simulink library "casper_library_accumulators"  (Simulink 7.2)
settings: Solver=ode45  SolverMode=SingleTasking  StartTime=0.0  StopTime=10.0  RelTol=1e-3
values from neighbouring files (symbols this model uses):
  blockCountBits = ceil(log2(numBlocks))    [address_gen_vacc_v2_mask.m]
  blockRowBits = 0    [address_gen_vacc_v2_mask.m]
  comp = compi    [bus_accumulator_init.m]    (also in bus_addsub_init.m = comp*2; bus_convert_init.m; bus_logical_init.m = comp*2; bus_maddsub_init.m = max([compa, compb, compc]))
libraries: xbsIndex_r4 x698, xbsReplacements_r4 x61, casper_library_misc x17, xps_library x9
(part 3 of 5)

== system casper_library_accumulators/dram_vacc/ctrl_unit ==
  valid_data : Inport
  sync : Inport  Port=2
  en_RB_addr : Inport  Port=3
  Concat1 : xbsIndex_r4/Concat  num_inputs=3  dbl_ovrd=off  block_type=concat
      settings: block_version=9.2.01
  Convert2 : xbsIndex_r4/Convert  gui_display_data_type=Fixed-point  arith_type=Unsigned  n_bits=30  bin_pt=0  float_type=Single  exp_bits=8  fraction_bits=24  quantization=Truncate  overflow=Wrap  en=off  latency=0  dbl_ovrd=off  pipeline=off  block_type=convert
      settings: xl_area=[0, 0, 0, 0, 0, 0, 0]  block_version=9.2.01
  Delay1 : xbsIndex_r4/Delay  rst=off  infoeditControl=Selection of Reset will increase slice count due to use of real FFs and instead of SRLs  en=off  latency=2  dbl_ovrd=off  reg_retiming=on  block_type=delay
      settings: xl_area=[0, 0, 0, 0, 0, 0, 0]  block_version=9.2.01
  Delay2 : xbsIndex_r4/Delay  rst=off  infoeditControl=Selection of Reset will increase slice count due to use of real FFs and instead of SRLs  en=off  latency=1  dbl_ovrd=off  reg_retiming=on  block_type=delay
      settings: xl_area=[0, 0, 0, 0, 0, 0, 0]  block_version=9.2.01
  Mux : xbsIndex_r4/Mux  inputs=2  en=off  latency=0  precision=Full  arith_type="Signed  (2's comp)"  n_bits=8  bin_pt=2  quantization=Truncate  overflow=Wrap  dbl_ovrd=off  block_type=mux
      settings: xl_area=[0, 0, 0, 0, 0, 0, 0]  block_version=9.2.01
  Mux2 : xbsIndex_r4/Mux  inputs=2  en=off  latency=0  precision=Full  arith_type="Signed  (2's comp)"  n_bits=8  bin_pt=2  quantization=Truncate  overflow=Wrap  dbl_ovrd=off  block_type=mux
      settings: xl_area=[0, 0, 0, 0, 0, 0, 0]  block_version=9.2.01
  RB_active_or_finish : Subsystem
  address_gen_vacc_DRAM : Subsystem  mask{acc_length=acc_length, valid_length=burst_length}
      mask prompts: acc_length "Accumulation length?"; valid_length "Valid period length?"
      mask init:
      | address_gen_vacc_v2_mask;
  cmd_gen : Subsystem
  latch_rb_enable : Subsystem
  negedge : Subsystem
  readback_address_dram_vacc : Subsystem  mask{acc_length=acc_length, valid_length=valid_length}
      mask prompts: acc_length "Accumulation length?"; valid_length "Valid period length?"
      mask init:
      | readback_address_dram_vacc_mask;
  warn period Delay10 : xbsReplacements_r4/Warning  SystemSampleTime=-1  period=1
  warn period Delay20 : xbsReplacements_r4/Warning  SystemSampleTime=-1  period=1
  address : Outport
  cmd_tag : Outport  Port=2
  RB_active : Outport  Port=3
  RWn : Outport  Port=4
  cmd_valid : Outport  Port=5
  ready : Outport  Port=6
  wires:
  latch_rb_enable/2(cmd_tag) -> Concat1/3
  Delay1/1 -> latch_rb_enable/1(sync), readback_address_dram_vacc/1(sync)  "v"
  negedge/1(out) -> latch_rb_enable/3(negedge)
  latch_rb_enable/1(inc_addr_en) -> RB_active_or_finish/1(enable_rb_addr), readback_address_dram_vacc/2(en)
  readback_address_dram_vacc/1(readback_addr) -> Mux2/3
  valid_data/1 -> cmd_gen/1(valid_data)
  cmd_gen/6(rb_addr_en) -> negedge/1(in), Concat1/1, Mux2/1
  cmd_gen/5(ready) -> ready/1
  cmd_gen/4(cmd_valid) -> cmd_valid/1
  cmd_gen/3(RWn) -> Mux/1, RWn/1
  RB_active_or_finish/1(rb_active) -> RB_active/1
  Mux2/1 -> address/1, Convert2/1
  en_RB_addr/1 -> latch_rb_enable/2(rb_addr_enable)
  Delay2/1 -> address_gen_vacc_DRAM/1(sync)
  Concat1/1 -> cmd_tag/1
  Convert2/1 -> Concat1/2
  cmd_gen/2(wr_addr_en) -> address_gen_vacc_DRAM/3(write_en)
  cmd_gen/1(re_addr_en) -> address_gen_vacc_DRAM/2(read_en)
  Mux/1 -> Mux2/2
  address_gen_vacc_DRAM/2(read_addr) -> Mux/3
  address_gen_vacc_DRAM/1(write_addr) -> Mux/2
  sync/1 -> Delay2/1, RB_active_or_finish/2(sync), Delay1/1, cmd_gen/2(sync)

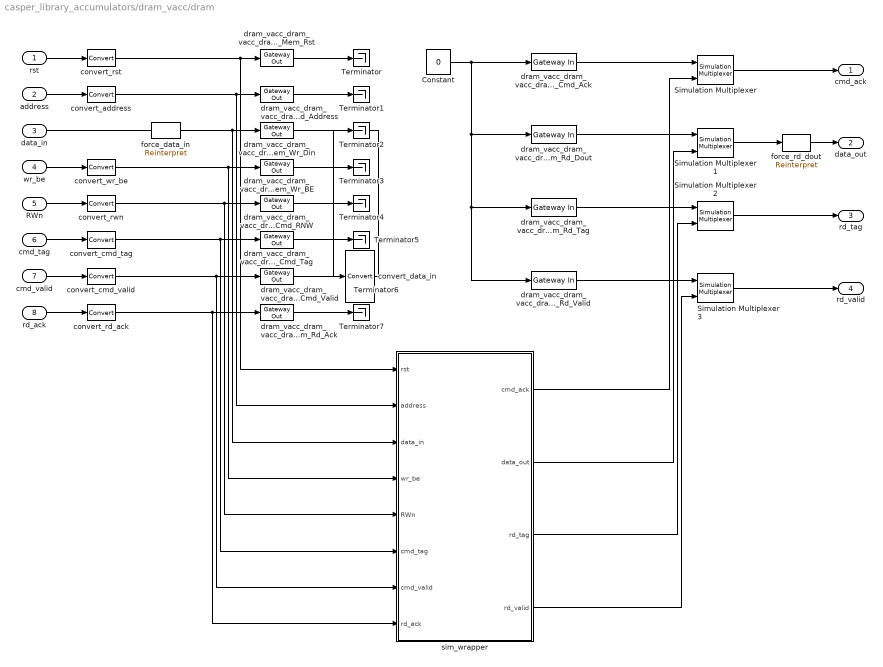
== system casper_library_accumulators/dram_vacc/dram ==
  rst : Inport
  address : Inport  Port=2
  data_in : Inport  Port=3
  wr_be : Inport  Port=4
  RWn : Inport  Port=5
  cmd_tag : Inport  Port=6
  cmd_valid : Inport  Port=7
  rd_ack : Inport  Port=8
  Constant : Constant  Value=0
  Simulation Multiplexer{,1..3} (4 alike) : xbsIndex_r4/Simulation Multiplexer  sim_sel=2  hw_sel=1  block_type=simmux
      settings: infoedit="Distinguish input subsystems as \"simulation only\" and \"generation only\".  The input specified For Simulation will be used during Simulink simulation.  The input specified For Generation will be used during code generation.  This block will typically be used on the output of a HW Co-Simulation, Black Box, or ModelSim subsystem.<P><P>Hardware Notes: This block costs nothing."  block_version=9.2.01
  Terminator{,1..7} (8 alike) : Terminator
  convert_address : xbsIndex_r4/Convert  gui_display_data_type=Fixed-point  arith_type=Unsigned  n_bits=32  bin_pt=0  float_type=Single  exp_bits=8  fraction_bits=24  quantization=Truncate  overflow=Wrap  en=off  latency=0  dbl_ovrd=off  pipeline=off  block_type=convert
      settings: xl_area=[0, 0, 0, 0, 0, 0, 0]  block_version=9.2.01
  convert_cmd_tag : xbsIndex_r4/Convert  gui_display_data_type=Fixed-point  arith_type=Unsigned  n_bits=32  bin_pt=0  float_type=Single  exp_bits=8  fraction_bits=24  quantization=Truncate  overflow=Wrap  en=off  latency=0  dbl_ovrd=off  pipeline=off  block_type=convert
      settings: xl_area=[0, 0, 0, 0, 0, 0, 0]  block_version=9.2.01
  convert_cmd_valid : xbsIndex_r4/Convert  gui_display_data_type=Fixed-point  arith_type=Unsigned  n_bits=1  bin_pt=0  float_type=Single  exp_bits=8  fraction_bits=24  quantization=Truncate  overflow=Wrap  en=off  latency=0  dbl_ovrd=off  pipeline=off  block_type=convert
      settings: xl_area=[0, 0, 0, 0, 0, 0, 0]  block_version=9.2.01
  convert_data_in : xbsIndex_r4/Convert  gui_display_data_type=Fixed-point  arith_type=Unsigned  n_bits=144  bin_pt=0  float_type=Single  exp_bits=8  fraction_bits=24  quantization=Truncate  overflow=Wrap  en=off  latency=0  dbl_ovrd=off  pipeline=off  block_type=convert
      settings: xl_area=[0, 0, 0, 0, 0, 0, 0]  block_version=9.2.01
  convert_rd_ack : xbsIndex_r4/Convert  gui_display_data_type=Fixed-point  arith_type=Unsigned  n_bits=1  bin_pt=0  float_type=Single  exp_bits=8  fraction_bits=24  quantization=Truncate  overflow=Wrap  en=off  latency=0  dbl_ovrd=off  pipeline=off  block_type=convert
      settings: xl_area=[0, 0, 0, 0, 0, 0, 0]  block_version=9.2.01
  convert_rst : xbsIndex_r4/Convert  gui_display_data_type=Fixed-point  arith_type=Unsigned  n_bits=1  bin_pt=0  float_type=Single  exp_bits=8  fraction_bits=24  quantization=Truncate  overflow=Wrap  en=off  latency=0  dbl_ovrd=off  pipeline=off  block_type=convert
      settings: xl_area=[0, 0, 0, 0, 0, 0, 0]  block_version=9.2.01
  convert_rwn : xbsIndex_r4/Convert  gui_display_data_type=Fixed-point  arith_type=Unsigned  n_bits=1  bin_pt=0  float_type=Single  exp_bits=8  fraction_bits=24  quantization=Truncate  overflow=Wrap  en=off  latency=0  dbl_ovrd=off  pipeline=off  block_type=convert
      settings: xl_area=[0, 0, 0, 0, 0, 0, 0]  block_version=9.2.01
  convert_wr_be : xbsIndex_r4/Convert  gui_display_data_type=Fixed-point  arith_type=Unsigned  n_bits=18  bin_pt=0  float_type=Single  exp_bits=8  fraction_bits=24  quantization=Truncate  overflow=Wrap  en=off  latency=0  dbl_ovrd=off  pipeline=off  block_type=convert
      settings: xl_area=[0, 0, 0, 0, 0, 0, 0]  block_version=9.2.01
  dram_vacc_dram_vacc_dram_Mem_Cmd_Ack : xbsIndex_r4/Gateway In  gui_display_data_type=Fixed-point  arith_type=Unsigned  n_bits=1  bin_pt=0  preci_type=Single  exp_width=8  frac_width=24  quantization=Truncate  overflow=Wrap  period=sample_period  dbl_ovrd=off  timing_constraint=None  locs_specified=off  LOCs={}  hdl_port=on  block_type=gatewayin
      settings: infoedit="Gateway in block.  Converts inputs of type Simulink integer, double and fixed point to  Xilinx fixed point type.<P><P>Hardware notes:  In hardware these blocks become top level input ports."  xl_area=[0, 0, 0, 0, 0, 0, 0]  block_version=9.2.01
  dram_vacc_dram_vacc_dram_Mem_Cmd_Address : xbsIndex_r4/Gateway Out  hdl_port=on  timing_constraint=None  locs_specified=off  LOCs={}  block_type=gatewayout
      settings: infoedit="Gateway out block.  Converts Xilinx fixed point inputs into ouputs of type Simulink integer, double, or fixed point.<P><P>Hardware notes:  In hardware these blocks become top level output ports or are discarded, depending on how they are configured."  xl_area=[0, 0, 0, 0, 0, 0, 0]  block_version=9.2.01
  dram_vacc_dram_vacc_dram_Mem_Cmd_RNW : xbsIndex_r4/Gateway Out  hdl_port=on  timing_constraint=None  locs_specified=off  LOCs={}  block_type=gatewayout
      settings: infoedit="Gateway out block.  Converts Xilinx fixed point inputs into ouputs of type Simulink integer, double, or fixed point.<P><P>Hardware notes:  In hardware these blocks become top level output ports or are discarded, depending on how they are configured."  xl_area=[0, 0, 0, 0, 0, 0, 0]  block_version=9.2.01
  dram_vacc_dram_vacc_dram_Mem_Cmd_Tag : xbsIndex_r4/Gateway Out  hdl_port=on  timing_constraint=None  locs_specified=off  LOCs={}  block_type=gatewayout
      settings: infoedit="Gateway out block.  Converts Xilinx fixed point inputs into ouputs of type Simulink integer, double, or fixed point.<P><P>Hardware notes:  In hardware these blocks become top level output ports or are discarded, depending on how they are configured."  xl_area=[0, 0, 0, 0, 0, 0, 0]  block_version=9.2.01
  dram_vacc_dram_vacc_dram_Mem_Cmd_Valid : xbsIndex_r4/Gateway Out  hdl_port=on  timing_constraint=None  locs_specified=off  LOCs={}  block_type=gatewayout
      settings: infoedit="Gateway out block.  Converts Xilinx fixed point inputs into ouputs of type Simulink integer, double, or fixed point.<P><P>Hardware notes:  In hardware these blocks become top level output ports or are discarded, depending on how they are configured."  xl_area=[0, 0, 0, 0, 0, 0, 0]  block_version=9.2.01
  dram_vacc_dram_vacc_dram_Mem_Rd_Ack : xbsIndex_r4/Gateway Out  hdl_port=on  timing_constraint=None  locs_specified=off  LOCs={}  block_type=gatewayout
      settings: infoedit="Gateway out block.  Converts Xilinx fixed point inputs into ouputs of type Simulink integer, double, or fixed point.<P><P>Hardware notes:  In hardware these blocks become top level output ports or are discarded, depending on how they are configured."  xl_area=[0, 0, 0, 0, 0, 0, 0]  block_version=9.2.01
  dram_vacc_dram_vacc_dram_Mem_Rd_Dout : xbsIndex_r4/Gateway In  gui_display_data_type=Fixed-point  arith_type=Unsigned  n_bits=144  bin_pt=0  preci_type=Single  exp_width=8  frac_width=24  quantization=Truncate  overflow=Wrap  period=sample_period  dbl_ovrd=off  timing_constraint=None  locs_specified=off  LOCs={}  hdl_port=on  block_type=gatewayin
      settings: infoedit="Gateway in block.  Converts inputs of type Simulink integer, double and fixed point to  Xilinx fixed point type.<P><P>Hardware notes:  In hardware these blocks become top level input ports."  xl_area=[0, 0, 0, 0, 0, 0, 0]  block_version=9.2.01
  dram_vacc_dram_vacc_dram_Mem_Rd_Tag : xbsIndex_r4/Gateway In  gui_display_data_type=Fixed-point  arith_type=Unsigned  n_bits=32  bin_pt=0  preci_type=Single  exp_width=8  frac_width=24  quantization=Truncate  overflow=Wrap  period=sample_period  dbl_ovrd=off  timing_constraint=None  locs_specified=off  LOCs={}  hdl_port=on  block_type=gatewayin
      settings: infoedit="Gateway in block.  Converts inputs of type Simulink integer, double and fixed point to  Xilinx fixed point type.<P><P>Hardware notes:  In hardware these blocks become top level input ports."  xl_area=[0, 0, 0, 0, 0, 0, 0]  block_version=9.2.01
  dram_vacc_dram_vacc_dram_Mem_Rd_Valid : xbsIndex_r4/Gateway In  gui_display_data_type=Fixed-point  arith_type=Unsigned  n_bits=1  bin_pt=0  preci_type=Single  exp_width=8  frac_width=24  quantization=Truncate  overflow=Wrap  period=sample_period  dbl_ovrd=off  timing_constraint=None  locs_specified=off  LOCs={}  hdl_port=on  block_type=gatewayin
      settings: infoedit="Gateway in block.  Converts inputs of type Simulink integer, double and fixed point to  Xilinx fixed point type.<P><P>Hardware notes:  In hardware these blocks become top level input ports."  xl_area=[0, 0, 0, 0, 0, 0, 0]  block_version=9.2.01
  dram_vacc_dram_vacc_dram_Mem_Rst : xbsIndex_r4/Gateway Out  hdl_port=on  timing_constraint=None  locs_specified=off  LOCs={}  block_type=gatewayout
      settings: infoedit="Gateway out block.  Converts Xilinx fixed point inputs into ouputs of type Simulink integer, double, or fixed point.<P><P>Hardware notes:  In hardware these blocks become top level output ports or are discarded, depending on how they are configured."  xl_area=[0, 0, 0, 0, 0, 0, 0]  block_version=9.2.01
  dram_vacc_dram_vacc_dram_Mem_Wr_BE : xbsIndex_r4/Gateway Out  hdl_port=on  timing_constraint=None  locs_specified=off  LOCs={}  block_type=gatewayout
      settings: infoedit="Gateway out block.  Converts Xilinx fixed point inputs into ouputs of type Simulink integer, double, or fixed point.<P><P>Hardware notes:  In hardware these blocks become top level output ports or are discarded, depending on how they are configured."  xl_area=[0, 0, 0, 0, 0, 0, 0]  block_version=9.2.01
  dram_vacc_dram_vacc_dram_Mem_Wr_Din : xbsIndex_r4/Gateway Out  hdl_port=on  timing_constraint=None  locs_specified=off  LOCs={}  block_type=gatewayout
      settings: infoedit="Gateway out block.  Converts Xilinx fixed point inputs into ouputs of type Simulink integer, double, or fixed point.<P><P>Hardware notes:  In hardware these blocks become top level output ports or are discarded, depending on how they are configured."  xl_area=[0, 0, 0, 0, 0, 0, 0]  block_version=9.2.01
  force_data_in : xbsIndex_r4/Reinterpret  force_arith_type=on  arith_type=Unsigned  force_bin_pt=on  bin_pt=0  block_type=reinterpret
      settings: infoedit="Changes signal type without altering the binary representation.   You can changed the signal between signed and unsigned, and relocate the binary point.<P><P>Hardware notes: In hardware this block costs nothing.<P><P>Example:  Suppose the input is 6 bits wide, signed, with 2 fractional bits, and the output is forced to unsigned with 0 fractional bits.  Then an input of -2.0 (1110.00 in binary 2's complement) becomes an output of 56 (111000 in binary)."  block_version=9.2.01
  force_rd_dout : xbsIndex_r4/Reinterpret  force_arith_type=on  arith_type=Unsigned  force_bin_pt=on  bin_pt=0  block_type=reinterpret
      settings: infoedit="Changes signal type without altering the binary representation.   You can changed the signal between signed and unsigned, and relocate the binary point.<P><P>Hardware notes: In hardware this block costs nothing.<P><P>Example:  Suppose the input is 6 bits wide, signed, with 2 fractional bits, and the output is forced to unsigned with 0 fractional bits.  Then an input of -2.0 (1110.00 in binary 2's complement) becomes an output of 56 (111000 in binary)."  block_version=9.2.01
  sim_wrapper : Subsystem
  cmd_ack : Outport
  data_out : Outport  Port=2
  rd_tag : Outport  Port=3
  rd_valid : Outport  Port=4
  wires:
  force_rd_dout/1 -> data_out/1
  force_data_in/1 -> dram_vacc_dram_vacc_dram_Mem_Wr_Din/1, sim_wrapper/3(data_in)
  convert_rd_ack/1 -> dram_vacc_dram_vacc_dram_Mem_Rd_Ack/1, sim_wrapper/8(rd_ack)
  convert_cmd_valid/1 -> dram_vacc_dram_vacc_dram_Mem_Cmd_Valid/1, sim_wrapper/7(cmd_valid)
  convert_cmd_tag/1 -> dram_vacc_dram_vacc_dram_Mem_Cmd_Tag/1, sim_wrapper/6(cmd_tag)
  convert_rwn/1 -> dram_vacc_dram_vacc_dram_Mem_Cmd_RNW/1, sim_wrapper/5(RWn)
  convert_wr_be/1 -> dram_vacc_dram_vacc_dram_Mem_Wr_BE/1, sim_wrapper/4(wr_be)
  convert_data_in/1 -> force_data_in/1
  convert_address/1 -> dram_vacc_dram_vacc_dram_Mem_Cmd_Address/1, sim_wrapper/2(address)
  convert_rst/1 -> dram_vacc_dram_vacc_dram_Mem_Rst/1, sim_wrapper/1(rst)
  rd_ack/1 -> convert_rd_ack/1
  cmd_valid/1 -> convert_cmd_valid/1
  cmd_tag/1 -> convert_cmd_tag/1
  RWn/1 -> convert_rwn/1
  data_in/1 -> convert_data_in/1
  rst/1 -> convert_rst/1
  address/1 -> convert_address/1
  wr_be/1 -> convert_wr_be/1
  dram_vacc_dram_vacc_dram_Mem_Rst/1 -> Terminator/1
  dram_vacc_dram_vacc_dram_Mem_Cmd_Address/1 -> Terminator1/1
  dram_vacc_dram_vacc_dram_Mem_Wr_Din/1 -> Terminator2/1
  dram_vacc_dram_vacc_dram_Mem_Wr_BE/1 -> Terminator3/1
  dram_vacc_dram_vacc_dram_Mem_Cmd_RNW/1 -> Terminator4/1
  dram_vacc_dram_vacc_dram_Mem_Cmd_Tag/1 -> Terminator5/1
  dram_vacc_dram_vacc_dram_Mem_Cmd_Valid/1 -> Terminator6/1
  dram_vacc_dram_vacc_dram_Mem_Rd_Ack/1 -> Terminator7/1
  Constant/1 -> dram_vacc_dram_vacc_dram_Mem_Cmd_Ack/1, dram_vacc_dram_vacc_dram_Mem_Rd_Dout/1, dram_vacc_dram_vacc_dram_Mem_Rd_Tag/1, dram_vacc_dram_vacc_dram_Mem_Rd_Valid/1
  dram_vacc_dram_vacc_dram_Mem_Cmd_Ack/1 -> Simulation Multiplexer/1
  Simulation Multiplexer/1 -> cmd_ack/1
  dram_vacc_dram_vacc_dram_Mem_Rd_Dout/1 -> Simulation Multiplexer1/1
  Simulation Multiplexer1/1 -> force_rd_dout/1
  Simulation Multiplexer2/1 -> rd_tag/1
  Simulation Multiplexer3/1 -> rd_valid/1
  dram_vacc_dram_vacc_dram_Mem_Rd_Tag/1 -> Simulation Multiplexer2/1
  dram_vacc_dram_vacc_dram_Mem_Rd_Valid/1 -> Simulation Multiplexer3/1
  sim_wrapper/1(cmd_ack) -> Simulation Multiplexer/2
  sim_wrapper/2(data_out) -> Simulation Multiplexer1/2
  sim_wrapper/3(rd_tag) -> Simulation Multiplexer2/2
  sim_wrapper/4(rd_valid) -> Simulation Multiplexer3/2

== system casper_library_accumulators/dram_vacc/fifo_empty_check ==
  cmd_valid : Inport
  tag_in : Inport  Port=2
  RWn : Inport  Port=3
  dram_data_tag : Inport  Port=4
  rd_ack : Inport  Port=5
  rd_valid : Inport  Port=6
  Convert : xbsIndex_r4/Convert  gui_display_data_type=Fixed-point  arith_type=Boolean  n_bits=8  bin_pt=6  float_type=Single  exp_bits=8  fraction_bits=24  quantization=Truncate  overflow=Wrap  en=off  latency=0  dbl_ovrd=off  pipeline=off  block_type=convert
      settings: xl_area=[0, 0, 0, 0, 0, 0, 0]  block_version=9.2.01
  Counter : xbsIndex_r4/Counter  cnt_type=Free Running  cnt_to=Inf  operation=Up  start_count=0  cnt_by_val=1  arith_type=Unsigned  n_bits=1  bin_pt=0  load_pin=off  rst=off  en=on  explicit_period=off  period=1  dbl_ovrd=off  use_behavioral_HDL=on  implementation=Fabric  use_rpm=on  block_type=counter
      settings: xl_area=[0, 0, 0, 0, 0, 0, 0]  block_version=9.2.01
  Delay1 : xbsIndex_r4/Delay  rst=off  infoeditControl=Selection of Reset will increase slice count due to use of real FFs and instead of SRLs  en=off  latency=1  dbl_ovrd=off  reg_retiming=on  block_type=delay
      settings: xl_area=[0, 0, 0, 0, 0, 0, 0]  block_version=9.2.01
  Delay2 : xbsIndex_r4/Delay  rst=off  infoeditControl=Selection of Reset will increase slice count due to use of real FFs and instead of SRLs  en=off  latency=1  dbl_ovrd=off  reg_retiming=on  block_type=delay
      settings: xl_area=[0, 0, 0, 0, 0, 0, 0]  block_version=9.2.01
  Logical : xbsIndex_r4/Logical  logical_function=AND  inputs=2  en=off  latency=0  precision=Full  arith_type=Unsigned  n_bits=8  bin_pt=2  align_bp=on  dbl_ovrd=off  block_type=logical
      settings: xl_area=[0, 0, 0, 0, 0, 0, 0]  block_version=9.2.01
  Logical1 : xbsIndex_r4/Logical  logical_function=AND  inputs=3  en=off  latency=0  precision=Full  arith_type=Unsigned  n_bits=8  bin_pt=2  align_bp=on  dbl_ovrd=off  block_type=logical
      settings: xl_area=[0, 0, 0, 0, 0, 0, 0]  block_version=9.2.01
  Logical2 : xbsIndex_r4/Logical  logical_function=AND  inputs=2  en=off  latency=0  precision=Full  arith_type=Unsigned  n_bits=8  bin_pt=2  align_bp=on  dbl_ovrd=off  block_type=logical
      settings: xl_area=[0, 0, 0, 0, 0, 0, 0]  block_version=9.2.01
  Register1 : xbsIndex_r4/Register  init=0  rst=on  en=on  dbl_ovrd=off  block_type=register
      settings: xl_area=[0, 0, 0, 0, 0, 0, 0]  block_version=9.2.01
  Relational : xbsIndex_r4/Relational  mode=a=b  en=off  latency=1  dbl_ovrd=off  block_type=relational
      settings: xl_area=[0, 0, 0, 0, 0, 0, 0]  block_version=9.2.01
  Relational1 : xbsIndex_r4/Relational  mode=a!=b  en=on  latency=1  dbl_ovrd=off  block_type=relational
      settings: xl_area=[0, 0, 0, 0, 0, 0, 0]  block_version=9.2.01
  last_read_tag : xbsIndex_r4/Register  init=0  rst=off  en=on  dbl_ovrd=off  block_type=register
      settings: xl_area=[0, 0, 0, 0, 0, 0, 0]  block_version=9.2.01
  negedge : Subsystem
  warn period Logical10 : xbsReplacements_r4/Warning  SystemSampleTime=-1  period=1
  warn period Register10 : xbsReplacements_r4/Warning  SystemSampleTime=-1  period=1
  warn period Relational10 : xbsReplacements_r4/Warning  SystemSampleTime=-1  period=1
  done : Outport
  wires:
  Logical2/1 -> Register1/2
  Convert/1 -> Register1/1, Register1/3
  Register1/1 -> done/1
  negedge/1(out) -> Convert/1
  Relational1/1 -> Logical2/1
  Counter/1 -> negedge/1(in)
  Logical1/1 -> Counter/1
  Relational/1 -> Logical1/1
  Delay1/1 -> Logical1/2
  rd_ack/1 -> Delay1/1
  Delay2/1 -> Logical1/3
  rd_valid/1 -> Delay2/1
  dram_data_tag/1 -> Relational/2
  last_read_tag/1 -> Relational/1, Relational1/2
  Logical/1 -> last_read_tag/2, Logical2/2, Relational1/3
  tag_in/1 -> last_read_tag/1, Relational1/1
  RWn/1 -> Logical/2
  cmd_valid/1 -> Logical/1

== system casper_library_accumulators/dsp48e_bram_vacc/delay_bram ==
  In1 : Inport
  Constant2 : xbsIndex_r4/Constant  const=1  gui_display_data_type=Fixed-point  arith_type=Boolean  n_bits=1  bin_pt=0  preci_type=Single  exp_width=8  frac_width=24  explicit_period=on  period=1  equ=P=C  opselect=C  inp2=PCIN>>17  opr=+  inp1=P  carry=CIN  dbl_ovrd=off  block_type=constant
  Counter : xbsIndex_r4/Counter  cnt_type=Count Limited  cnt_to=DelayLen - bram_latency - 1  operation=Up  start_count=0  cnt_by_val=1  arith_type=Unsigned  n_bits=BitWidth  bin_pt=0  load_pin=off  rst=off  en=off  explicit_period=off  period=1  dbl_ovrd=off  use_behavioral_HDL=on  implementation=Fabric  use_rpm=off  block_type=counter
      settings: xl_area=[0, 0, 0, 0, 0, 0, 0]
  Single Port RAM : xbsIndex_r4/Single Port RAM  depth=2^BitWidth  initVector=0  distributed_mem=Block RAM  write_mode=Read Before Write  rst=off  init_reg=0  en=off  latency=bram_latency  dbl_ovrd=off  optimize=Area  use_rpm=off  block_type=spram
      settings: xl_area=[0, 0, 0, 0, 0, 0, 0]  block_version=10.1.3
  Out1 : Outport
  wires:
  Single Port RAM/1 -> Out1/1
  Counter/1 -> Single Port RAM/1
  In1/1 -> Single Port RAM/2
  Constant2/1 -> Single Port RAM/3

== system casper_library_accumulators/dsp48e_bram_vacc/pulse_ext ==
  in : Inport
  Constant5 : xbsIndex_r4/Constant  const=pulse_len  gui_display_data_type=Fixed-point  arith_type=Unsigned  n_bits=bits  bin_pt=0  preci_type=Single  exp_width=8  frac_width=24  explicit_period=off  period=1  equ=P=C  opselect=C  inp2=PCIN>>17  opr=+  inp1=P  carry=CIN  dbl_ovrd=off  block_type=constant
  Counter3 : xbsIndex_r4/Counter  cnt_type=Free Running  cnt_to=1023  operation=Up  start_count=0  cnt_by_val=1  arith_type=Unsigned  n_bits=bits  bin_pt=0  load_pin=off  rst=on  en=on  explicit_period=on  period=1  dbl_ovrd=off  use_behavioral_HDL=on  implementation=Fabric  use_rpm=on  block_type=counter
      settings: xl_area=[0, 0, 0, 0, 0, 0, 0]
  Relational5 : xbsIndex_r4/Relational  mode=a!=b  en=off  latency=0  dbl_ovrd=off  block_type=relational
      settings: xl_area=[0, 0, 0, 0, 0, 0, 0]  block_version=10.1.3
  posedge : Subsystem  Tag=Rising Edge Detector
  out : Outport
  wires:
  posedge/1(Out) -> Counter3/1
  in/1 -> posedge/1(In)
  Relational5/1 -> out/1, Counter3/2
  Constant5/1 -> Relational5/2
  Counter3/1 -> Relational5/1

== system casper_library_accumulators/qdr_vacc/acc ==
  a : Inport
  b : Inport  Port=2
  blank_b : Inport  Port=3
  AddSub4 : xbsIndex_r4/AddSub  mode=Addition  use_carryin=off  use_carryout=off  en=off  latency=2  precision=User Defined  arith_type="Signed  (2's comp)"  n_bits=4  bin_pt=0  quantization="Round  (unbiased: +/- Inf)"  overflow=Wrap  dbl_ovrd=off  use_behavioral_HDL=on  hw_selection=Fabric  pipelined=on  use_rpm=on  block_type=addsub
      settings: xl_area=[0, 0, 0, 0, 0, 0, 0]  block_version=9.2.01
  AddSub5 : xbsIndex_r4/AddSub  mode=Addition  use_carryin=off  use_carryout=off  en=off  latency=2  precision=User Defined  arith_type="Signed  (2's comp)"  n_bits=32  bin_pt=0  quantization="Round  (unbiased: +/- Inf)"  overflow=Wrap  dbl_ovrd=off  use_behavioral_HDL=on  hw_selection=Fabric  pipelined=on  use_rpm=on  block_type=addsub
      settings: xl_area=[0, 0, 0, 0, 0, 0, 0]  block_version=9.2.01
  Concat1v1 : xbsIndex_r4/Concat  num_inputs=2  dbl_ovrd=off  block_type=concat
      settings: block_version=9.2.01
  Constant3 : xbsIndex_r4/Constant  const=0  gui_display_data_type=Fixed-point  arith_type=Unsigned  n_bits=36  bin_pt=0  preci_type=Single  exp_width=8  frac_width=24  explicit_period=on  period=1  equ=P=C  opselect=C  inp2=PCIN>>17  opr=+  inp1=P  carry=CIN  dbl_ovrd=off  block_type=constant
      settings: block_version=9.2.01
  Reinterpret{,1,4..5} (4 alike) : xbsIndex_r4/Reinterpret  force_arith_type=on  arith_type="Signed  (2's comp)"  force_bin_pt=on  bin_pt=0  block_type=reinterpret
      settings: infoedit="Changes signal type without altering the binary representation.   You can changed the signal between signed and unsigned, and relocate the binary point.<P><P>Hardware notes: In hardware this block costs nothing.<P><P>Example:  Suppose the input is 6 bits wide, signed, with 2 fractional bits, and the output is forced to unsigned with 0 fractional bits.  Then an input of -2.0 (1110.00 in binary 2's complement) becomes an output of 56 (111000 in binary)."  block_version=9.2.01
  Reinterpret8 : xbsIndex_r4/Reinterpret  force_arith_type=on  arith_type=Unsigned  force_bin_pt=on  bin_pt=0  block_type=reinterpret
      settings: infoedit="Changes signal type without altering the binary representation.   You can changed the signal between signed and unsigned, and relocate the binary point.<P><P>Hardware notes: In hardware this block costs nothing.<P><P>Example:  Suppose the input is 6 bits wide, signed, with 2 fractional bits, and the output is forced to unsigned with 0 fractional bits.  Then an input of -2.0 (1110.00 in binary 2's complement) becomes an output of 56 (111000 in binary)."  block_version=9.2.01
  Reinterpret9 : xbsIndex_r4/Reinterpret  force_arith_type=on  arith_type=Unsigned  force_bin_pt=on  bin_pt=0  block_type=reinterpret
      settings: infoedit="Changes signal type without altering the binary representation.   You can changed the signal between signed and unsigned, and relocate the binary point.<P><P>Hardware notes: In hardware this block costs nothing.<P><P>Example:  Suppose the input is 6 bits wide, signed, with 2 fractional bits, and the output is forced to unsigned with 0 fractional bits.  Then an input of -2.0 (1110.00 in binary 2's complement) becomes an output of 56 (111000 in binary)."  block_version=9.2.01
  Slice1 : xbsIndex_r4/Slice  nbits=4  boolean_output=off  mode=Lower Bit Location + Width  bit1=96  base1=MSB of Input  bit0=32  base0=LSB of Input  dbl_ovrd=off  block_type=slice
      settings: infoedit="Extracts a given range of bits from each input sample and presents it at the output.  The output type is ordinarily unsigned with binary point at zero, but can be Boolean when the slice is one bit wide.<P><P>Hardware notes: In hardware this block costs nothing."  block_version=9.2.01
  Slice15 : xbsIndex_r4/Slice  nbits=4  boolean_output=off  mode=Lower Bit Location + Width  bit1=96  base1=MSB of Input  bit0=32  base0=LSB of Input  dbl_ovrd=off  block_type=slice
      settings: infoedit="Extracts a given range of bits from each input sample and presents it at the output.  The output type is ordinarily unsigned with binary point at zero, but can be Boolean when the slice is one bit wide.<P><P>Hardware notes: In hardware this block costs nothing."  block_version=9.2.01
  Slice16 : xbsIndex_r4/Slice  nbits=32  boolean_output=off  mode=Lower Bit Location + Width  bit1=-32  base1=MSB of Input  bit0=0  base0=LSB of Input  dbl_ovrd=off  block_type=slice
      settings: infoedit="Extracts a given range of bits from each input sample and presents it at the output.  The output type is ordinarily unsigned with binary point at zero, but can be Boolean when the slice is one bit wide.<P><P>Hardware notes: In hardware this block costs nothing."  block_version=9.2.01
  Slice2 : xbsIndex_r4/Slice  nbits=32  boolean_output=off  mode=Lower Bit Location + Width  bit1=-32  base1=MSB of Input  bit0=0  base0=LSB of Input  dbl_ovrd=off  block_type=slice
      settings: infoedit="Extracts a given range of bits from each input sample and presents it at the output.  The output type is ordinarily unsigned with binary point at zero, but can be Boolean when the slice is one bit wide.<P><P>Hardware notes: In hardware this block costs nothing."  block_version=9.2.01
  rd_addr_sel : xbsIndex_r4/Mux  inputs=2  en=off  latency=0  precision=Full  arith_type=Unsigned  n_bits=16  bin_pt=14  quantization=Truncate  overflow=Wrap  dbl_ovrd=off  block_type=mux
  Out : Outport
  wires:
  Constant3/1 -> rd_addr_sel/3
  blank_b/1 -> rd_addr_sel/1
  rd_addr_sel/1 -> Slice1/1, Slice2/1
  b/1 -> rd_addr_sel/2
  AddSub5/1 -> Reinterpret9/1
  Reinterpret5/1 -> AddSub5/2
  Slice2/1 -> Reinterpret5/1
  Slice16/1 -> Reinterpret1/1
  Reinterpret1/1 -> AddSub5/1
  Reinterpret9/1 -> Concat1v1/2
  Concat1v1/1 -> Out/1
  a/1 -> Slice16/1, Slice15/1
  AddSub4/1 -> Reinterpret8/1
  Reinterpret4/1 -> AddSub4/2
  Slice1/1 -> Reinterpret4/1
  Slice15/1 -> Reinterpret/1
  Reinterpret/1 -> AddSub4/1
  Reinterpret8/1 -> Concat1v1/1

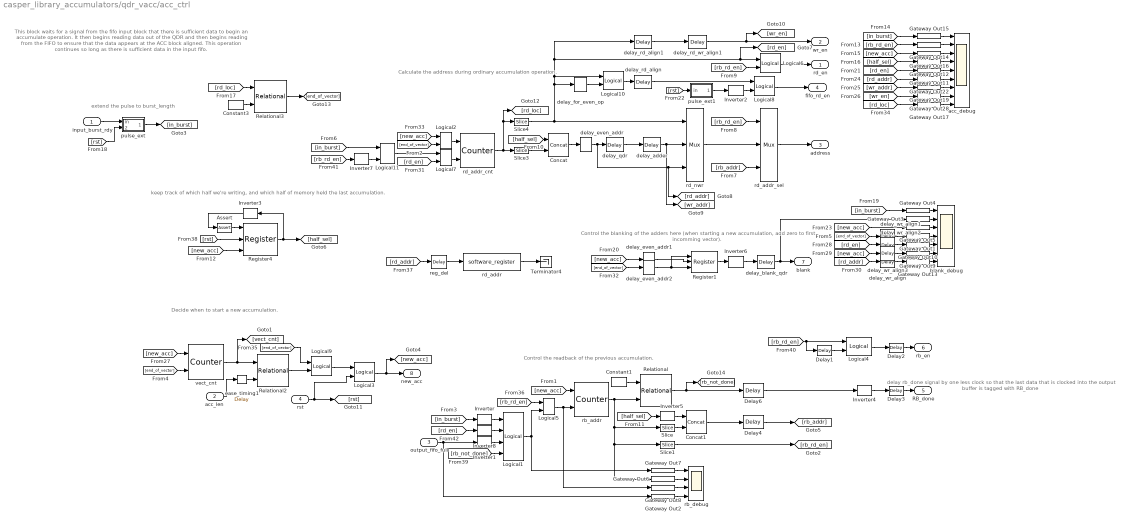
== system casper_library_accumulators/qdr_vacc/acc_ctrl ==
  note: extend the pulse to
      | burst_length
  note: This block waits for a signal from the
      | fifo input block that there is sufficient data
      | to begin an accumulate operation.
      |
      | It then begins reading data out of the QDR and
      | then begins reading from the FIFO to ensure
      | that the data appears at the ACC block aligned.
      |
      | This operation continues so long as there is
      | sufficient data in the input fifo.
  note: keep track of which half we're writing,
      | and which half of memory
      | held the last accumulation.
  note: delay rb_done signal by
      | one less clock so that the last
      | data that is clocked into
      | the output buffer is tagged with RB_done
  note: Control the readback of the
      | previous accumulation.
  note: Control the blanking of the
      | adders here (when starting a
      | new accumulation, add zero
      | to first incomming vector).
  note: Calculate the address during ordinary
      | accumulation operation.
  note: Decide when to start a new accumulation.
  input_burst_rdy : Inport
  acc_len : Inport  Port=2
  output_fifo_full : Inport  Port=3
  rst : Inport  Port=4
  Assert : xbsIndex_r4/Assert  assert_type=on  type_source=Explicitly  gui_display_data_type=Fixed-point  arith_type=Unsigned  n_bits=1  bin_pt=0  preci_type=Single  exp_width=8  frac_width=24  assert_rate=on  rate_source=Explicitly  period=1  output_port=on  block_type=assert
      settings: infoedit=Asserts a user-defined sample rate and/or type on a signal.<P><P>Hardware notes: In hardware this block costs nothing.  block_version=10.1.3
  Concat : xbsIndex_r4/Concat  num_inputs=2  dbl_ovrd=off  block_type=concat
      settings: block_version=10.1.3
  Concat1 : xbsIndex_r4/Concat  num_inputs=2  dbl_ovrd=off  block_type=concat
      settings: block_version=10.1.3
  Constant1 : xbsIndex_r4/Constant  const=vector_len - 1  gui_display_data_type=Fixed-point  arith_type=Unsigned  n_bits=vector_bits  bin_pt=0  preci_type=Single  exp_width=8  frac_width=24  explicit_period=on  period=1  equ=P=C  opselect=C  inp2=PCIN>>17  opr=+  inp1=P  carry=CIN  dbl_ovrd=off  block_type=constant
  Constant3 : xbsIndex_r4/Constant  const=vector_len-1  gui_display_data_type=Fixed-point  arith_type=Unsigned  n_bits=vector_bits  bin_pt=0  preci_type=Single  exp_width=8  frac_width=24  explicit_period=on  period=1  equ=P=C  opselect=C  inp2=PCIN>>17  opr=+  inp1=P  carry=CIN  dbl_ovrd=off  block_type=constant
  Delay1 : xbsIndex_r4/Delay  rst=off  infoeditControl=Selection of Reset will increase slice count due to use of real FFs and instead of SRLs  en=off  latency=1  dbl_ovrd=off  reg_retiming=on  block_type=delay
  Delay2 : xbsIndex_r4/Delay  rst=off  infoeditControl=Selection of Reset will increase slice count due to use of real FFs and instead of SRLs  en=off  latency=delay_qdr  dbl_ovrd=off  reg_retiming=on  block_type=delay
  Delay3 : xbsIndex_r4/Delay  rst=off  infoeditControl=Selection of Reset will increase slice count due to use of real FFs and instead of SRLs  en=off  latency=delay_qdr-1  dbl_ovrd=off  reg_retiming=on  block_type=delay
  Delay4 : xbsIndex_r4/Delay  rst=off  infoeditControl=Selection of Reset will increase slice count due to use of real FFs and instead of SRLs  en=off  latency=1  dbl_ovrd=off  reg_retiming=on  block_type=delay
  Delay6 : xbsIndex_r4/Delay  rst=off  infoeditControl=Selection of Reset will increase slice count due to use of real FFs and instead of SRLs  en=off  latency=1  dbl_ovrd=off  reg_retiming=on  block_type=delay
  Gateway Out{1..17,19,22,28} (20 alike) : xbsIndex_r4/Gateway Out  hdl_port=off  timing_constraint=None  locs_specified=off  LOCs={}  block_type=gatewayout
      settings: infoedit="Gateway out block.  Converts Xilinx fixed point inputs into ouputs of type Simulink integer, double, or fixed point.<P><P>Hardware notes:  In hardware these blocks become top level output ports or are discarded, depending on how they are configured."  xl_area=[0, 0, 0, 0, 0, 0, 0]  block_version=10.1.3
  Inverter{,1..2,4..8} (8 alike) : xbsIndex_r4/Inverter  en=off  latency=0  dbl_ovrd=off  block_type=inv
  Inverter3 : xbsIndex_r4/Inverter  Orientation=left  en=off  latency=0  dbl_ovrd=off  block_type=inv
  Logical1 : xbsIndex_r4/Logical  logical_function=AND  inputs=4  en=off  latency=0  precision=Full  arith_type=Unsigned  n_bits=16  bin_pt=0  align_bp=on  dbl_ovrd=off  block_type=logical
  Logical{2..7,10} (7 alike) : xbsIndex_r4/Logical  logical_function=OR  inputs=2  en=off  latency=0  precision=Full  arith_type=Unsigned  n_bits=16  bin_pt=0  align_bp=on  dbl_ovrd=off  block_type=logical
  Logical11 : xbsIndex_r4/Logical  logical_function=AND  inputs=2  en=off  latency=0  precision=Full  arith_type=Unsigned  n_bits=16  bin_pt=0  align_bp=on  dbl_ovrd=off  block_type=logical
  Logical8 : xbsIndex_r4/Logical  logical_function=AND  inputs=2  en=off  latency=0  precision=Full  arith_type=Unsigned  n_bits=16  bin_pt=0  align_bp=on  dbl_ovrd=off  block_type=logical
  Logical9 : xbsIndex_r4/Logical  logical_function=AND  inputs=2  en=off  latency=0  precision=Full  arith_type=Unsigned  n_bits=16  bin_pt=0  align_bp=on  dbl_ovrd=off  block_type=logical
  Register1 : xbsIndex_r4/Register  init=0  rst=on  en=on  dbl_ovrd=off  block_type=register
  Register4 : xbsIndex_r4/Register  init=0  rst=on  en=on  dbl_ovrd=off  block_type=register
  Relational : xbsIndex_r4/Relational  mode=a>=b  en=off  latency=0  dbl_ovrd=off  block_type=relational
      settings: block_version=10.1.3
  Relational2 : xbsIndex_r4/Relational  mode=a>=b  en=off  latency=0  dbl_ovrd=off  block_type=relational
      settings: block_version=10.1.3
  Relational3 : xbsIndex_r4/Relational  mode=a>=b  en=off  latency=0  dbl_ovrd=off  block_type=relational
      settings: block_version=10.1.3
  Slice : xbsIndex_r4/Slice  nbits=vector_bits-1  boolean_output=off  mode=Lower Bit Location + Width  bit1=0  base1=MSB of Input  bit0=1  base0=LSB of Input  dbl_ovrd=off  block_type=slice
      settings: infoedit="Extracts a given range of bits from each input sample and presents it at the output.  The output type is ordinarily unsigned with binary point at zero, but can be Boolean when the slice is one bit wide.<P><P>Hardware notes: In hardware this block costs nothing."  block_version=10.1.3
  Slice1 : xbsIndex_r4/Slice  nbits=1  boolean_output=on  mode=Lower Bit Location + Width  bit1=-1  base1=MSB of Input  bit0=0  base0=LSB of Input  dbl_ovrd=off  block_type=slice
      settings: infoedit="Extracts a given range of bits from each input sample and presents it at the output.  The output type is ordinarily unsigned with binary point at zero, but can be Boolean when the slice is one bit wide.<P><P>Hardware notes: In hardware this block costs nothing."  block_version=10.1.3
  Slice3 : xbsIndex_r4/Slice  nbits=1  boolean_output=off  mode=Two Bit Locations  bit1=0  base1=MSB of Input  bit0=1  base0=LSB of Input  dbl_ovrd=off  block_type=slice
      settings: infoedit="Extracts a given range of bits from each input sample and presents it at the output.  The output type is ordinarily unsigned with binary point at zero, but can be Boolean when the slice is one bit wide.<P><P>Hardware notes: In hardware this block costs nothing."  block_version=10.1.3
  Slice4 : xbsIndex_r4/Slice  nbits=1  boolean_output=on  mode=Lower Bit Location + Width  bit1=-1  base1=MSB of Input  bit0=0  base0=LSB of Input  dbl_ovrd=off  block_type=slice
      settings: infoedit="Extracts a given range of bits from each input sample and presents it at the output.  The output type is ordinarily unsigned with binary point at zero, but can be Boolean when the slice is one bit wide.<P><P>Hardware notes: In hardware this block costs nothing."  block_version=10.1.3
  Terminator4 : Terminator
  acc_debug : Scope  NumInputPorts=9
      settings: TimeRange=10000  YMin=0~-1~-1~0.95~0~500~500~0~-5  YMax=1~1~1~1.05~1~1100~1100~1~5  SaveName=ScopeData5
  blank_debug : Scope  NumInputPorts=7
      settings: TimeRange=10000  YMin=0~1~-1~-1~0~-1~50  YMax=1~1~1~1~1~1~250  SaveName=ScopeData6
  delay_adder : xbsIndex_r4/Delay  rst=off  infoeditControl=Selection of Reset will increase slice count due to use of real FFs and instead of SRLs  en=off  latency=delay_adder  dbl_ovrd=off  reg_retiming=on  block_type=delay
  delay_blank_qdr : xbsIndex_r4/Delay  rst=off  infoeditControl=Selection of Reset will increase slice count due to use of real FFs and instead of SRLs  en=off  latency=delay_qdr  dbl_ovrd=off  reg_retiming=on  block_type=delay
  delay_even_addr : xbsIndex_r4/Delay  rst=off  infoeditControl=Selection of Reset will increase slice count due to use of real FFs and instead of SRLs  en=off  latency=1  dbl_ovrd=off  reg_retiming=on  block_type=delay
  delay_even_addr1 : xbsIndex_r4/Delay  rst=off  infoeditControl=Selection of Reset will increase slice count due to use of real FFs and instead of SRLs  en=off  latency=1  dbl_ovrd=off  reg_retiming=on  block_type=delay
  delay_even_addr2 : xbsIndex_r4/Delay  rst=off  infoeditControl=Selection of Reset will increase slice count due to use of real FFs and instead of SRLs  en=off  latency=1  dbl_ovrd=off  reg_retiming=on  block_type=delay
  delay_for_even_op : xbsIndex_r4/Delay  rst=off  infoeditControl=Selection of Reset will increase slice count due to use of real FFs and instead of SRLs  en=off  latency=1  dbl_ovrd=off  reg_retiming=on  block_type=delay
  delay_qdr : xbsIndex_r4/Delay  rst=off  infoeditControl=Selection of Reset will increase slice count due to use of real FFs and instead of SRLs  en=off  latency=delay_qdr  dbl_ovrd=off  reg_retiming=on  block_type=delay
  delay_rd_align : xbsIndex_r4/Delay  rst=off  infoeditControl=Selection of Reset will increase slice count due to use of real FFs and instead of SRLs  en=off  latency=delay_qdr-delay_in_fifo  dbl_ovrd=off  reg_retiming=on  block_type=delay
  delay_rd_align1 : xbsIndex_r4/Delay  rst=off  infoeditControl=Selection of Reset will increase slice count due to use of real FFs and instead of SRLs  en=off  latency=delay_qdr  dbl_ovrd=off  reg_retiming=on  block_type=delay
  delay_rd_wr_align1 : xbsIndex_r4/Delay  rst=off  infoeditControl=Selection of Reset will increase slice count due to use of real FFs and instead of SRLs  en=off  latency=delay_adder  dbl_ovrd=off  reg_retiming=on  block_type=delay
  delay_wr_align{,1..3} (4 alike) : xbsIndex_r4/Delay  rst=off  infoeditControl=Selection of Reset will increase slice count due to use of real FFs and instead of SRLs  en=off  latency=delay_qdr  dbl_ovrd=off  reg_retiming=on  block_type=delay
  ease_timing1 : xbsIndex_r4/Delay  rst=off  infoeditControl=Selection of Reset will increase slice count due to use of real FFs and instead of SRLs  en=off  latency=1  dbl_ovrd=off  reg_retiming=on  block_type=delay
  pulse_ext : Subsystem  AncestorBlock=casper_library_misc/pulse_ext  mask(pulse_ext){pulse_len=burst_len}
      mask prompts: pulse_len "Length of Pulse"
      mask help:
      | Extends a boolean signal to be high for the specified number of clocks after
      | the last high input.
      mask init:
      | bits = ceil(log2(pulse_len+1));
      mask Help: eval('xlWeb(''http://casper.berkeley.edu/wiki/Pulse_ext'')')
  pulse_ext1 : Subsystem  AncestorBlock=casper_library_misc/pulse_ext  mask(pulse_ext){pulse_len=delay_qdr-delay_in_fifo}
      mask prompts: pulse_len "Length of Pulse"
      mask help:
      | Extends a boolean signal to be high for the specified number of clocks after
      | the last high input.
      mask init:
      | bits = ceil(log2(pulse_len+1));
      mask Help: eval('xlWeb(''http://casper.berkeley.edu/wiki/Pulse_ext'')')
  rb_addr : xbsIndex_r4/Counter  cnt_type=Free Running  cnt_to=Inf  operation=Up  start_count=0  cnt_by_val=1  arith_type=Unsigned  n_bits=vector_bits  bin_pt=0  load_pin=off  rst=on  en=on  explicit_period=on  period=1  dbl_ovrd=off  use_behavioral_HDL=on  implementation=Fabric  use_rpm=off  block_type=counter
  rb_debug : Scope  NumInputPorts=4
      settings: TimeRange=10000  YMin=0~0~0~0  YMax=1~1000~1~1  SaveName=ScopeData5
  rd_addr : xps_library/software_register  Tag=xps:sw_reg  SystemSampleTime=-1  io_dir=To Processor  arith_type=Unsigned  bitwidth=32  bin_pt=0  sample_period=1  gw_name=casper_library_accumulators_qdr_vacc_acc_ctrl_rd_addr_user_data_in
  rd_addr_cnt : xbsIndex_r4/Counter  cnt_type=Free Running  cnt_to=vector_len-1  operation=Up  start_count=0  cnt_by_val=1  arith_type=Unsigned  n_bits=vector_bits  bin_pt=0  load_pin=off  rst=on  en=on  explicit_period=on  period=1  dbl_ovrd=off  use_behavioral_HDL=on  implementation=Fabric  use_rpm=off  block_type=counter
  rd_addr_sel : xbsIndex_r4/Mux  inputs=2  en=off  latency=0  precision=Full  arith_type=Unsigned  n_bits=16  bin_pt=14  quantization=Truncate  overflow=Wrap  dbl_ovrd=off  block_type=mux
  rd_nwr : xbsIndex_r4/Mux  inputs=2  en=off  latency=0  precision=Full  arith_type=Unsigned  n_bits=16  bin_pt=14  quantization=Truncate  overflow=Wrap  dbl_ovrd=off  block_type=mux
  reg_del : xbsIndex_r4/Delay  rst=off  infoeditControl=Selection of Reset will increase slice count due to use of real FFs and instead of SRLs  en=off  latency=1  dbl_ovrd=off  reg_retiming=on  block_type=delay
  vect_cnt : xbsIndex_r4/Counter  cnt_type=Free Running  cnt_to=Inf  operation=Up  start_count=1  cnt_by_val=1  arith_type=Unsigned  n_bits=32  bin_pt=0  load_pin=off  rst=on  en=on  explicit_period=on  period=1  dbl_ovrd=off  use_behavioral_HDL=on  implementation=Fabric  use_rpm=off  block_type=counter
  rd_en : Outport
  wr_en : Outport  Port=2
  address : Outport  Port=3
  fifo_rd_en : Outport  Port=4
  RB_done : Outport  Port=5
  rb_en : Outport  Port=6
  blank : Outport  Port=7
  new_acc : Outport  Port=8
  wires:
  Inverter8/1 -> Logical1/2
  [rd_en] -> Inverter8/1
  Inverter7/1 -> Logical11/2
  [rb_not_done] -> Logical1/4
  Inverter1/1 -> Logical1/3
  Inverter/1 -> Logical1/1
  [in_burst] -> Logical11/1
  [rb_rd_en] -> Inverter7/1
  [rb_rd_en] -> Logical5/1
  [rb_rd_en] -> Delay1/1, Logical4/1
  delay_for_even_op/1 -> Logical10/2
  Logical10/1 -> delay_rd_align/1
  pulse_ext1/1(out) -> Inverter2/1
  Inverter2/1 -> Logical8/2
  [rst] -> pulse_ext1/1(in)
  Logical8/1 -> fifo_rd_en/1
  delay_rd_align/1 -> Logical8/1
  [rd_addr] -> reg_del/1
  reg_del/1 -> rd_addr/1
  rd_addr/1 -> Terminator4/1
  [rst] -> Register4/2
  [new_acc] -> Register4/3
  delay_even_addr2/1 -> Register1/3, Register1/1
  delay_even_addr1/1 -> Register1/2
  delay_even_addr/1 -> delay_qdr/1, rd_nwr/3, [rd_addr]
  Slice1/1 -> [rb_rd_en]
  [end_of_vector] -> Logical9/1
  Logical9/1 -> Logical3/1
  Relational2/1 -> Logical9/2
  Gateway Out17/1 -> acc_debug/9
  [rd_loc] -> Gateway Out17/1
  delay_wr_align2/1 -> Gateway Out10/1
  delay_wr_align3/1 -> Gateway Out9/1
  delay_wr_align1/1 -> Gateway Out1/1
  Inverter6/1 -> delay_blank_qdr/1
  [new_acc] -> Logical2/1
  [end_of_vector] -> Logical2/2
  Logical2/1 -> rd_addr_cnt/1
  [end_of_vector] -> delay_wr_align1/1
  [new_acc] -> delay_even_addr1/1
  [end_of_vector] -> delay_even_addr2/1
  [end_of_vector] -> vect_cnt/2
  [rd_en] -> Logical7/2
  Logical11/1 -> Logical7/1
  Logical7/1 -> rd_addr_cnt/2
  Slice3/1 -> Concat/2
  Gateway Out13/1 -> blank_debug/7
  delay_wr_align/1 -> Gateway Out13/1
  [rd_addr] -> delay_wr_align/1
  [new_acc] -> delay_wr_align3/1
  [rd_en] -> delay_wr_align2/1
  Gateway Out9/1 -> blank_debug/6
  Gateway Out10/1 -> blank_debug/5
  Gateway Out7/1 -> rb_debug/1
  Gateway Out6/1 -> rb_debug/2
  Gateway Out8/1 -> rb_debug/3
  Gateway Out2/1 -> rb_debug/4
  [rst] -> pulse_ext/2(rst)
  Slice4/1 -> Logical10/1, delay_rd_align1/1, Logical6/1, [rd_en], delay_for_even_op/1, rd_nwr/1
  input_burst_rdy/1 -> pulse_ext/1(in)
  pulse_ext/1(out) -> [in_burst]
  rd_addr_cnt/1 -> [rd_loc], Slice4/1, Slice3/1
  delay_qdr/1 -> delay_adder/1
  delay_adder/1 -> rd_nwr/2, [wr_addr]
  Relational/1 -> [rb_not_done], Delay6/1
  [new_acc] -> rb_addr/1
  output_fifo_full/1 -> Gateway Out2/1, Inverter1/1
  Delay2/1 -> rb_en/1
  Logical6/1 -> rd_en/1
  [in_burst] -> Inverter/1
  [rb_rd_en] -> rd_addr_sel/1
  rd_nwr/1 -> rd_addr_sel/2
  [rb_rd_en] -> Logical6/2
  rd_addr_sel/1 -> address/1
  Register4/1 -> Inverter3/1, [half_sel]
  Inverter3/1 -> Assert/1
  Assert/1 -> Register4/1
  Gateway Out15/1 -> acc_debug/1
  Gateway Out14/1 -> acc_debug/2
  Gateway Out16/1 -> acc_debug/3
  Gateway Out12/1 -> acc_debug/4
  Gateway Out11/1 -> acc_debug/5
  [rb_rd_en] -> Gateway Out14/1
  [in_burst] -> Gateway Out15/1
  [new_acc] -> Gateway Out16/1
  [half_sel] -> Gateway Out12/1
  Register1/1 -> Inverter6/1
  Gateway Out4/1 -> blank_debug/1
  Gateway Out3/1 -> blank_debug/2
  Gateway Out5/1 -> blank_debug/3
  [in_burst] -> Gateway Out4/1
  [new_acc] -> Gateway Out5/1
  [rd_en] -> Gateway Out11/1
  Gateway Out22/1 -> acc_debug/6
  Gateway Out19/1 -> acc_debug/7
  [rd_addr] -> Gateway Out22/1
  [wr_addr] -> Gateway Out19/1
  acc_len/1 -> ease_timing1/1
  vect_cnt/1 -> [vect_cnt], Relational2/1
  [rd_loc] -> Relational3/1
  Constant3/1 -> Relational3/2
  Relational3/1 -> [end_of_vector]
  delay_blank_qdr/1 -> blank/1, Gateway Out3/1
  [wr_en] -> Gateway Out28/1
  Gateway Out28/1 -> acc_debug/8
  rst/1 -> Logical3/2, [rst]
  Logical3/1 -> new_acc/1, [new_acc]
  [new_acc] -> vect_cnt/1
  ease_timing1/1 -> Relational2/2
  Delay3/1 -> RB_done/1
  [half_sel] -> Concat/1
  Concat/1 -> delay_even_addr/1
  [half_sel] -> Inverter5/1
  Inverter5/1 -> Concat1/1
  [rb_addr] -> rd_addr_sel/3
  Concat1/1 -> Delay4/1
  Slice/1 -> Concat1/2
  Constant1/1 -> Relational/1
  rb_addr/1 -> Slice1/1, Gateway Out6/1, Slice/1, Relational/2
  Inverter4/1 -> Delay3/1
  Delay4/1 -> [rb_addr]
  delay_rd_align1/1 -> delay_rd_wr_align1/1
  delay_rd_wr_align1/1 -> wr_en/1, [wr_en]
  Logical1/1 -> Logical5/2, Gateway Out7/1
  Delay6/1 -> Inverter4/1
  Logical4/1 -> Delay2/1
  Delay1/1 -> Logical4/2
  Logical5/1 -> Gateway Out8/1, rb_addr/2
  Gateway Out1/1 -> blank_debug/4

== system casper_library_accumulators/simple_bram_vacc/delay_bram ==
  In1 : Inport
  Constant2 : xbsIndex_r4/Constant  const=1  gui_display_data_type=Fixed-point  arith_type=Boolean  n_bits=1  bin_pt=0  preci_type=Single  exp_width=8  frac_width=24  explicit_period=on  period=1  equ=P=C  opselect=C  inp2=PCIN>>17  opr=+  inp1=P  carry=CIN  dbl_ovrd=off  block_type=constant
  Counter : xbsIndex_r4/Counter  cnt_type=Count Limited  cnt_to=DelayLen - bram_latency - 1  operation=Up  start_count=0  cnt_by_val=1  arith_type=Unsigned  n_bits=BitWidth  bin_pt=0  load_pin=off  rst=off  en=off  explicit_period=off  period=1  dbl_ovrd=off  use_behavioral_HDL=on  implementation=Fabric  use_rpm=off  block_type=counter
      settings: xl_area=[0, 0, 0, 0, 0, 0, 0]
  Single Port RAM : xbsIndex_r4/Single Port RAM  depth=2^BitWidth  initVector=0  distributed_mem=Block RAM  write_mode=Read Before Write  rst=off  init_reg=0  en=off  latency=bram_latency  dbl_ovrd=off  optimize=Area  use_rpm=off  block_type=spram
      settings: xl_area=[0, 0, 0, 0, 0, 0, 0]  block_version=10.1.3
  Out1 : Outport
  wires:
  Single Port RAM/1 -> Out1/1
  Counter/1 -> Single Port RAM/1
  In1/1 -> Single Port RAM/2
  Constant2/1 -> Single Port RAM/3
